simulink model "slex3"  (R2018b)
settings: Solver=FixedStepAuto  StartTime=0.0  StopTime=10.0  FixedStep=0.01  RelTol=1e-3
settings Model: Creator=19810  LastModifiedBy=19810
settings DataIOCC: InspectSignalLogs=on

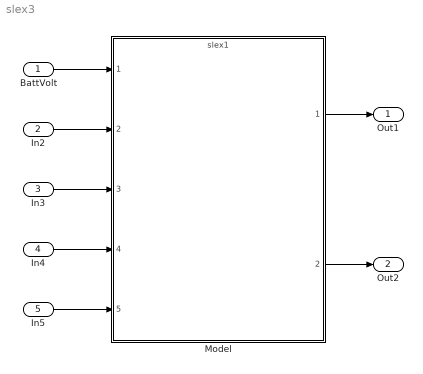
== system slex3 ==
  BattVolt : Inport
  In2 : Inport  Port=2
  In3 : Inport  Port=3
  In4 : Inport  Port=4
  In5 : Inport  Port=5
  Model : ModelReference  ModelNameDialog=slex1.slx  SimulationMode=Normal  ModelReferenceVersion=1.14
  Out1 : Outport
  Out2 : Outport  Port=2
  wires:
  BattVolt/1 -> Model/1
  In2/1 -> Model/2
  In3/1 -> Model/3
  In4/1 -> Model/4
  In5/1 -> Model/5
  Model/1 -> Out1/1
  Model/2 -> Out2/1
